simulink model "PMSM_Simulation_2025a"  (R2025a)
settings: Solver=FixedStepDiscrete  StartTime=0.0  StopTime=10  FixedStep=0.00005/200  RelTol=1e-3
values from neighbouring files (symbols this model uses):
  MC_DCurrLopKi_CFG = 0.008293758    [PMSM_MC_Data_2025a.sldd]
  MC_DCurrLopKp_CFG = 0.0870848    [PMSM_MC_Data_2025a.sldd]
  MC_MotModeDebug_CFG = 255.0    [PMSM_MC_Data_2025a.sldd]
  MC_POLE_NUM_CFG = 7.0    [PMSM_MC_Data_2025a.sldd]
  MC_QCurrLopKi_CFG = 0.008293758    [PMSM_MC_Data_2025a.sldd]
  MC_QCurrLopKp_CFG = 0.0870848    [PMSM_MC_Data_2025a.sldd]
  MC_SpdLopKi_CFG = 1.0E-5    [PMSM_MC_Data_2025a.sldd]
  MC_SpdLopKp_CFG = 0.002    [PMSM_MC_Data_2025a.sldd]
undefined symbols (not defined in the file or in its folder): Ls, magnitude, Rs
libraries: simulink x28, slpidlib x6, spsDCVoltageSourceLib x1, spsPermanentMagnetSynchronousMachineLib x1, spsUniversalBridgeLib x1, sps_lib x1
(part 3 of 3)

== system PMSM_Simulation_2025a/PMSM_MC/MC_HighFrqTask/FOC/SensorLessAlgorithm/SMO+Artan/SMO/LPF1 ==
  In : Inport
  TiCon : Inport  Port=2
  Add : Sum  Inputs=+-
  Add1 : Sum
  Constant : Constant  Value=single(1)
  Delay : Delay  DelayLength=1  InitialConditionSource=Input port
      settings: InputPortMap=u0,p4
  Product : Product
  Product1 : Product
  out : Outport
  wires:
  Delay/1 -> Product1/2
  Add1/1 -> out/1, Delay/1
  Product1/1 -> Add1/2
  Product/1 -> Add1/1
  Constant/1 -> Add/1
  Add/1 -> Product1/1
  TiCon/1 -> Product/2, Add/2
  In/1 -> Product/1, Delay/2

== system PMSM_Simulation_2025a/PMSM_MC/MC_HighFrqTask/FOC/SensorLessAlgorithm/SMO+Artan/SMO/Sat ==
  Err_now : Inport
  h : Inport  Port=2
  ErrMax : Inport  Port=3
  Constant : Constant
  Constant1 : Constant  Value=-1
  Divide : Product  Inputs=*/
  Gain : Gain  Gain=-1
  Product : Product
  Relational Operator : RelationalOperator  Operator=>  OutDataTypeStr=boolean  RndMeth=Simplest  InputSameDT=off
  Relational Operator1 : RelationalOperator  Operator=<  OutDataTypeStr=boolean  RndMeth=Simplest  InputSameDT=off
  Switch : Switch  Criteria=u2 ~= 0  SaturateOnIntegerOverflow=off  InputSameDT=off
  Switch1 : Switch  Criteria=u2 ~= 0  SaturateOnIntegerOverflow=off  InputSameDT=off
  AlphaE : Outport
  wires:
  Err_now/1 -> Divide/1, Relational Operator1/1, Relational Operator/1
  ErrMax/1 -> Divide/2, Gain/1, Relational Operator/2
  Relational Operator/1 -> Switch/2
  Constant/1 -> Switch/1
  Gain/1 -> Relational Operator1/2
  Relational Operator1/1 -> Switch1/2
  Switch1/1 -> Switch/3
  Constant1/1 -> Switch1/1
  Divide/1 -> Switch1/3
  Switch/1 -> Product/1
  h/1 -> Product/2
  Product/1 -> AlphaE/1

== system PMSM_Simulation_2025a/PMSM_MC/MC_HighFrqTask/FOC/SensorLessAlgorithm/SMO+Artan/SMO/Sat1 ==
  Err_now : Inport
  h : Inport  Port=2
  ErrMax : Inport  Port=3
  Constant : Constant
  Constant1 : Constant  Value=-1
  Divide : Product  Inputs=*/
  Gain : Gain  Gain=-1
  Product : Product
  Relational Operator : RelationalOperator  Operator=>  OutDataTypeStr=boolean  RndMeth=Simplest  InputSameDT=off
  Relational Operator1 : RelationalOperator  Operator=<  OutDataTypeStr=boolean  RndMeth=Simplest  InputSameDT=off
  Switch : Switch  Criteria=u2 ~= 0  SaturateOnIntegerOverflow=off  InputSameDT=off
  Switch1 : Switch  Criteria=u2 ~= 0  SaturateOnIntegerOverflow=off  InputSameDT=off
  AlphaE : Outport
  wires:
  Err_now/1 -> Divide/1, Relational Operator1/1, Relational Operator/1
  ErrMax/1 -> Divide/2, Gain/1, Relational Operator/2
  Relational Operator/1 -> Switch/2
  Constant/1 -> Switch/1
  Gain/1 -> Relational Operator1/2
  Relational Operator1/1 -> Switch1/2
  Switch1/1 -> Switch/3
  Constant1/1 -> Switch1/1
  Divide/1 -> Switch1/3
  Switch/1 -> Product/1
  h/1 -> Product/2
  Product/1 -> AlphaE/1

== system PMSM_Simulation_2025a/PMSM_MC/MC_HighFrqTask/FOC/SensorLessAlgorithm/SMO+PLL/PLL/LPF ==
  In : Inport
  TiCon : Inport  Port=2
  Add : Sum  Inputs=+-
  Add1 : Sum
  Constant : Constant  Value=single(1)
  Delay : Delay  DelayLength=1  InitialConditionSource=Input port
      settings: InputPortMap=u0,p4
  Product : Product
  Product1 : Product
  out : Outport
  wires:
  In/1 -> Delay/2, Product/1
  TiCon/1 -> Add/2, Product/2
  Add/1 -> Product1/1
  Constant/1 -> Add/1
  Product/1 -> Add1/1
  Product1/1 -> Add1/2
  Add1/1 -> Delay/1, out/1
  Delay/1 -> Product1/2

== system PMSM_Simulation_2025a/PMSM_MC/MC_HighFrqTask/FOC/SensorLessAlgorithm/SMO+PLL/SMO/LPF ==
  In : Inport
  TiCon : Inport  Port=2
  Add : Sum  Inputs=+-
  Add1 : Sum
  Constant : Constant  Value=single(1)
  Delay : Delay  DelayLength=1  InitialConditionSource=Input port
      settings: InputPortMap=u0,p4
  Product : Product
  Product1 : Product
  out : Outport
  wires:
  In/1 -> Delay/2, Product/1
  TiCon/1 -> Add/2, Product/2
  Add/1 -> Product1/1
  Constant/1 -> Add/1
  Product/1 -> Add1/1
  Product1/1 -> Add1/2
  Add1/1 -> Delay/1, out/1
  Delay/1 -> Product1/2

== system PMSM_Simulation_2025a/PMSM_MC/MC_HighFrqTask/FOC/SensorLessAlgorithm/SMO+PLL/SMO/LPF1 ==
  In : Inport
  TiCon : Inport  Port=2
  Add : Sum  Inputs=+-
  Add1 : Sum
  Constant : Constant  Value=single(1)
  Delay : Delay  DelayLength=1  InitialConditionSource=Input port
      settings: InputPortMap=u0,p4
  Product : Product
  Product1 : Product
  out : Outport
  wires:
  Delay/1 -> Product1/2
  Add1/1 -> out/1, Delay/1
  Product1/1 -> Add1/2
  Product/1 -> Add1/1
  Constant/1 -> Add/1
  Add/1 -> Product1/1
  TiCon/1 -> Product/2, Add/2
  In/1 -> Product/1, Delay/2

== system PMSM_Simulation_2025a/PMSM_MC/MC_HighFrqTask/FOC/SensorLessAlgorithm/SMO+PLL/SMO/Sat ==
  Err_now : Inport
  h : Inport  Port=2
  ErrMax : Inport  Port=3
  Constant : Constant
  Constant1 : Constant  Value=-1
  Divide : Product  Inputs=*/
  Gain : Gain  Gain=-1
  Product : Product
  Relational Operator : RelationalOperator  Operator=>  OutDataTypeStr=boolean  RndMeth=Simplest  InputSameDT=off
  Relational Operator1 : RelationalOperator  Operator=<  OutDataTypeStr=boolean  RndMeth=Simplest  InputSameDT=off
  Switch : Switch  Criteria=u2 ~= 0  SaturateOnIntegerOverflow=off  InputSameDT=off
  Switch1 : Switch  Criteria=u2 ~= 0  SaturateOnIntegerOverflow=off  InputSameDT=off
  AlphaE : Outport
  wires:
  Err_now/1 -> Divide/1, Relational Operator1/1, Relational Operator/1
  ErrMax/1 -> Divide/2, Gain/1, Relational Operator/2
  Relational Operator/1 -> Switch/2
  Constant/1 -> Switch/1
  Gain/1 -> Relational Operator1/2
  Relational Operator1/1 -> Switch1/2
  Switch1/1 -> Switch/3
  Constant1/1 -> Switch1/1
  Divide/1 -> Switch1/3
  Switch/1 -> Product/1
  h/1 -> Product/2
  Product/1 -> AlphaE/1

== system PMSM_Simulation_2025a/PMSM_MC/MC_HighFrqTask/FOC/SensorLessAlgorithm/SMO+PLL/SMO/Sat1 ==
  Err_now : Inport
  h : Inport  Port=2
  ErrMax : Inport  Port=3
  Constant : Constant
  Constant1 : Constant  Value=-1
  Divide : Product  Inputs=*/
  Gain : Gain  Gain=-1
  Product : Product
  Relational Operator : RelationalOperator  Operator=>  OutDataTypeStr=boolean  RndMeth=Simplest  InputSameDT=off
  Relational Operator1 : RelationalOperator  Operator=<  OutDataTypeStr=boolean  RndMeth=Simplest  InputSameDT=off
  Switch : Switch  Criteria=u2 ~= 0  SaturateOnIntegerOverflow=off  InputSameDT=off
  Switch1 : Switch  Criteria=u2 ~= 0  SaturateOnIntegerOverflow=off  InputSameDT=off
  AlphaE : Outport
  wires:
  Err_now/1 -> Divide/1, Relational Operator1/1, Relational Operator/1
  ErrMax/1 -> Divide/2, Gain/1, Relational Operator/2
  Relational Operator/1 -> Switch/2
  Constant/1 -> Switch/1
  Gain/1 -> Relational Operator1/2
  Relational Operator1/1 -> Switch1/2
  Switch1/1 -> Switch/3
  Constant1/1 -> Switch1/1
  Divide/1 -> Switch1/3
  Switch/1 -> Product/1
  h/1 -> Product/2
  Product/1 -> AlphaE/1

== stateflow chart PMSM_Simulation_2025a/PMSM_MC/MC_LowFrqTask/MotModeCtr/ModeMgr ==
  state RangeCheck [function]
    (default) -> (junction 21)
    (junction 21) -> (junction 23) [order 1] : [abs(MotOffsetBuff[0]-MotOffsetBuff[1])>100]
    (junction 21) -> (junction 24) [order 2] : {
        | MotCalNormal=1;
        | MotOffset = (MotOffsetBuff[0]+MotOffsetBuff[1])/2;
        | }
    (junction 23) -> (junction 25) : {MotCalNormal=0;}
    (junction 25) -> (junction 24)
    (junction 24) -> (junction 35)
  state SensorCtr
    state Calibrate
      state Init
        en:
        MotCtrMode=0;
      state Calibrate1
        en:
        MotCtrMode=1;
        MotCalThetae = 1.046;//60°
      state Calibrate2
        en:
        MotOffsetBuff[0]=Ecode_cnt-166;
        MotCtrMode=2;
        MotCalThetae = 2.093;//120°
      state RngChk
        en:
        MotOffsetBuff[1]=Ecode_cnt-333;
        RangeCheck();
      (default) -> Init
      Init -> Calibrate1 : [MotorSpdRef != 0]
      Calibrate1 -> Calibrate2 : [after(1.5,sec)]
      Calibrate2 -> RngChk : [after(1.5,sec)]
    state Normal
      state Stop
        en:
        MotCtrMode=4;
      state Run
        en:
        MotCtrMode=5;
      (default) -> SensorCtr.Normal.Stop
      SensorCtr.Normal.Run -> SensorCtr.Normal.Stop : [MotorSpdRef==0]
      SensorCtr.Normal.Stop -> SensorCtr.Normal.Run : [MotorSpdRef!=0]
    state CalFailed
      en:
      MotCtrMode=3;
    (default) -> Calibrate
    CalFailed -> Calibrate : [MotorSpdRef==0]
    RngChk -> CalFailed [order 1] : [MotCalNormal==0]
    RngChk -> Normal [order 2] : [MotCalNormal==1]
  state SensorLessCtr
    state Stop
      en:
      MotCtrMode=4;
    state StartFail
      en:
      MotCtrMode=6;
    state IFStart
      en:
      MotCtrMode=7;
    state Run
      en:
      MotCtrMode=5;
    (default) -> SensorLessCtr.Stop
    SensorLessCtr.Stop -> IFStart : [MotorSpdRef != 0]
    StartFail -> SensorLessCtr.Stop : [MotorSpdRef==0]
    SensorLessCtr.Run -> SensorLessCtr.Stop : [MotorSpdRef==0]
    IFStart -> StartFail [order 2] : [after(600,msec)]
    IFStart -> SensorLessCtr.Run [order 1] : [OLStartCompletedFlag==1]
  note: 注意此处的无感有感开环状态机
      | 的切换模式条件中，如果是仿真
      | 测试需要把速度设定改成不等于
      | 0，但是嵌入式模型部署中需要
      | 改成等于0
  state VFOpenLoop
    en:
    MotCtrMode = 8;
  (default) -> SensorCtr
  SensorCtr -> SensorLessCtr [order 1] : [//value is 1 mean sensorless control
      | SensorLessEn ==1 &&...
      | MotorSpdRef != 0]
  SensorLessCtr -> SensorCtr [order 1] : [//value is 0 mean sensor control
      | SensorLessEn ==0 &&...
      | MotorSpdRef != 0]
  SensorLessCtr -> VFOpenLoop [order 2] : [OpenLoopEn == 1&&...
      | MotorSpdRef != 0]
  VFOpenLoop -> SensorLessCtr [order 1] : [OpenLoopEn == 0&&...
      | MotorSpdRef != 0&&...
      | SensorLessEn == 1]
  VFOpenLoop -> SensorCtr [order 2] : [OpenLoopEn == 0&&...
      | MotorSpdRef != 0&&...
      | SensorLessEn == 0]
  SensorCtr -> VFOpenLoop [order 2] : [OpenLoopEn == 1&&...
      | MotorSpdRef != 0]
  data: MotCtrMode output uint8; Ecode_cnt input int32; MotorSpdRef input int16; MotOffset output int32; MotCalThetae output single; MotOffsetBuff local int32 size=2; MotCalNormal local boolean; SensorLessEn input boolean; OpenLoopEn input boolean; OLStartCompletedFlag input boolean

== stateflow chart PMSM_Simulation_2025a/PMSM_MC/MC_HighFrqTask/OpenLopMod/OpenLopThetaeCal ==
  state Stop
    en:
    //init output
    Thetae_SensLess = 0;
    OLStartCompletedFlag = 0;
    //init local variable
    WeRefRamped = 0;
    OLStableCnt = 0;
    TransmStep = 0;
    TransmFactor = 0;
    Thetae_OL = 0;
    note: 注意要给局部变量
        | 初始化赋值处理
  state VFOpenLoop
    state Align
      en:
      Thetae_SensLess = 0;
    state Open
      en,du:
      Ramping(OLWeRef,OLWeRampMaxStep);
      OLThetaeSum();
      Thetae_SensLess = Thetae_OL;
    (default) -> VFOpenLoop.Align
    VFOpenLoop.Align -> VFOpenLoop.Open : [after(100,msec)]
  state IFStart
    state Align
      en:
      Thetae_SensLess = 0;
    state Open
      en,du:
      Ramping(OLWeRef,OLWeRampMaxStep);
      OLThetaeSum();
      OLStableCntSum();
      Thetae_SensLess = Thetae_OL;
    note: TransmStep其实是根据切换时间算每次
        | 权重增加的步长，最终完成切换从0->1
    state Transm
      en:
      //cal steps according time
      TransmStep = 1/(OLWeightedTransmTime*1000/50);
      //transmite from open to close
      WeightedTransmite();
      du:
      WeightedTransmite();
    (default) -> IFStart.Align
    IFStart.Align -> IFStart.Open : [after(100,msec)]
    IFStart.Open -> Transm : [OLStableCnt>OLSpdStableCnt]
  state Ramping(in,MaxStep) [function]
    note: WeRefRamped指当前的局部真实被电机使用的一个设定递增速度值，电机最开始为0，当我的速度期望值比较大的时候，就会与现在WeRefRamped真实速度设定值比较，让他以MaxStep的递增速度累加或者累减，直到设定值与期望值的差值在[-MaxStep,+MaxStep]时，将当前速度赋值给定成期望值
    (default) -> (junction 23)
    (junction 23) -> (junction 30) [order 1] : [in - WeRefRamped > MaxStep]
    (junction 23) -> (junction 32) [order 2]
    (junction 30) -> (junction 41) : {
        | WeRefRamped = WeRefRamped + MaxStep;
        | }
    (junction 32) -> (junction 34) [order 1] : [in - WeRefRamped < -MaxStep]
    (junction 32) -> (junction 36) [order 2] : {
        | WeRefRamped = in;
        | }
    (junction 34) -> (junction 38) : {
        | WeRefRamped = WeRefRamped - MaxStep;
        | }
    (junction 38) -> (junction 36)
    (junction 41) -> (junction 38)
    (junction 36) -> (junction 43)
  state OLThetaeSum [function]
    note: MotCtrMode==8条件是为了VF开环使用的，
        | 我们的VF开环只进行正向累加，而MotorSpdRef
        | 主要用于IF启动的时候使用
    (default) -> (junction 28)
    (junction 28) -> (junction 48) [order 1] : [MotorSpdRef > 0||...
        | MotCtrMode == 8]
    (junction 28) -> (junction 52) [order 2] : {
        | Thetae_OL = Thetae_OL - WeRefRamped*Ts;
        | }
    (junction 48) -> (junction 50) : {
        | Thetae_OL = Thetae_OL + WeRefRamped*Ts;
        | }
    (junction 50) -> (junction 52)
    (junction 52) -> (junction 55)
    (junction 55) -> (junction 57) [order 1] : [Thetae_OL < 0]
    (junction 55) -> (junction 59) [order 2] : {
        | //set range to [0 2pi]
        | Thetae_OL = fmod(Thetae_OL,6.28);
        | }
    (junction 57) -> (junction 58) : {
        | //set range to [0 2pi]
        | Thetae_OL  = -Thetae_OL;
        | Thetae_OL = fmod(Thetae_OL,6.28);
        | Thetae_OL =  6.28 - Thetae_OL;
        | }
    (junction 58) -> (junction 59)
    (junction 59) -> (junction 60)
  state OLStableCntSum [function]
    note: 如果观测器速度大于设定的稳定速度就开始稳定计次
        | 如果出现速度小于阈值则计次再次为0
    (default) -> (junction 79)
    (junction 79) -> (junction 87) [order 1] : [(MotorSpdRef > 0 && Wm_Est>OLSpdStableThd) ||...
        | (MotorSpdRef < 0 && Wm_Est<-OLSpdStableThd)]
    (junction 79) -> (junction 85) [order 2] : {
        | OLStableCnt = 0;
        | }
    (junction 87) -> (junction 86) : {
        | OLStableCnt++;
        | }
    (junction 86) -> (junction 85)
    (junction 85) -> (junction 88)
  state WeightedTransmite [function]
    (default) -> (junction 103) : {
        | //update factor each sw cycle
        | TransmFactor = TransmFactor+TransmStep;
        | //open loop angle calculate
        | Ramping(OLWeRef,OLWeRampMaxStep);
        | OLThetaeSum();
        | }
    (junction 103) -> (junction 108) [order 1] : [TransmFactor>1]
    (junction 103) -> (junction 113) [order 2]
    (junction 108) -> (junction 111) : {
        | //limit to [0,1]
        | TransmFactor = 1;
        | }
    (junction 111) -> (junction 113)
    (junction 113) -> (junction 116)
    (junction 116) -> (junction 118) [order 1] : [TransmFactor>0.99]
    (junction 116) -> (junction 122) [order 2]
    (junction 118) -> (junction 120) : {
        | //开环切闭环完成
        | OLStartCompletedFlag = 1;
        | }
    (junction 120) -> (junction 122)
    (junction 122) -> (junction 125) : {
        | //计算一下输出的无感模式电角度
        | Thetae_SensLess = Thetae_OL*(1-TransmFactor) + Thetae_Est*TransmFactor;
        | }
  note: 加上MotCtrMode == 5条件判断的原因是由于速度环和电流环切换时序不一样，模式切换在低频任务中，为避免速度环和速度环积分影响，需要双条件判断
  state CloseLop
    en,du:
    Thetae_SensLess = Thetae_Est;
  (default) -> Stop
  Stop -> VFOpenLoop [order 1] : [MotCtrMode==8]
  VFOpenLoop -> Stop : [MotCtrMode!=8]
  Stop -> IFStart [order 2] : [MotCtrMode==7]
  CloseLop -> Stop : [MotCtrMode!=5]
  IFStart -> CloseLop : [OLStartCompletedFlag==1&&...
      | MotCtrMode==5]
  data: in function_input double; MaxStep function_input double; MotCtrMode input uint8; Wm_Est input single; Thetae_Est input single; MotorSpdRef input int16; OLWeRef input single; OLWeRampMaxStep input single; OLSpdStableThd input single; OLSpdStableCnt input single; Ts input single; Thetae_SensLess output single; OLStartCompletedFlag output boolean; WeRefRamped local single; OLWeightedTransmTime input single; Thetae_OL local single; OLStableCnt local uint16; TransmStep local single; TransmFactor local single

== stateflow chart PMSM_Simulation_2025a/Scheduler ==
  (default) -> (junction 6)
  (junction 6) -> (junction 11) [order 1] : [counter%%4000==3999]
  (junction 6) -> (junction 10) [order 2]
  (junction 11) -> (junction 9) : {trig_MidFrq_1ms;}
  (junction 9) -> (junction 10)
  (junction 10) -> (junction 36)
  (junction 36) -> (junction 38) [order 1] : [counter%%200==199]
  (junction 36) -> (junction 41) [order 2]
  (junction 38) -> (junction 40) : {trig_HighFrq_50us;}
  (junction 40) -> (junction 41)
  (junction 41) -> (junction 18)
  (junction 18) -> (junction 20) [order 1] : [counter>=100000000]
  (junction 18) -> (junction 24) [order 2] : {counter++;}
  (junction 20) -> (junction 22) : {counter=0;}
  (junction 22) -> (junction 24)
  (junction 24) -> (junction 27)
  data: counter local uint32 =0
  events: trig_MidFrq_1ms output FUNCTION_CALL_EVENT; trig_HighFrq_50us output FUNCTION_CALL_EVENT
